simulink model "KT_Robot_Robustness"  (R2025b)
settings: Solver=FixedStepDiscrete  StartTime=0.0  StopTime=tEnd  FixedStep=Ts  RelTol=1e-3
model workspace (MAT data in the model file):
  Ts = 0.05
  impact = [0; 0.1; 0.174532925199; 4; 1; 0.4; 0.04; -0.04; 2; 3.5]
  initialPose = [0; -0.6; 0]
  noise = [-0.649013765191 1.18116604197 -0.758453297284 -1.1096130385 -0.845551240008 -0.572664866458 -0.558680764474 0.17838022585 -0.196861446476 0.586442621667 -0.851886969622 0.800320709802 ... (7323 elements, 3x2441)]
  pathData = [0  0  0  4; 4  0  4  3; 4  3  7  4; 8  3  11  3; 8  6  14  0]
  robot = [0.05; 0.3; 12; 2]
  settings = [0.55; 0.5; 0.05; 1; 1.308996939; 2; 0; 0.12; 0.05; 2400]
  tEnd = 122
(part 1 of 2)
settings Model: Creator=ADMIN  LastModifiedBy=ADMIN
settings DataIOCC: SaveOutput=off  SaveTime=off

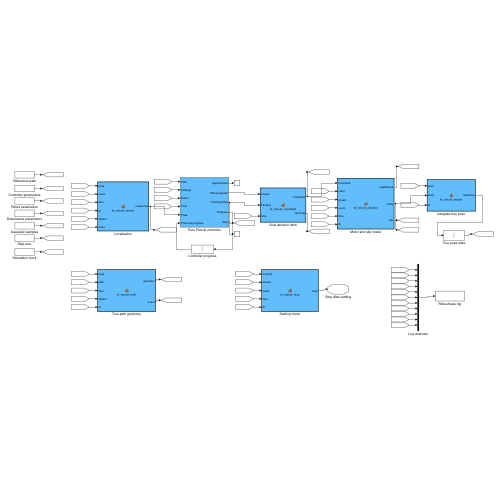
[thumbnail: Simulink's stored preview of the top-level diagram]
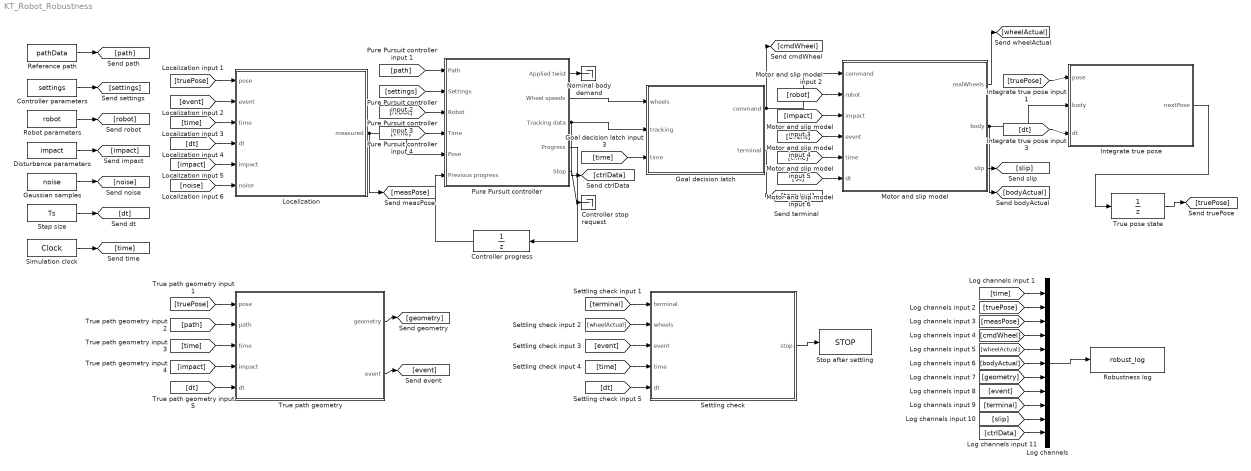
== system KT_Robot_Robustness ==
  Controller parameters : Constant  Value=settings
  Controller progress : UnitDelay  SampleTime=Ts  HasFrameUpgradeWarning=on
  Controller stop request : Terminator
  Disturbance parameters : Constant  Value=impact
  Gaussian samples : Constant  Value=noise
  Goal decision latch : MATLAB Function  TreatAsAtomicUnit=on
  Integrate true pose : MATLAB Function  TreatAsAtomicUnit=on
  Localization : MATLAB Function  TreatAsAtomicUnit=on
  Log channels : Mux  Inputs=[1 3 3 2 2 3 3 3 2 2 6]
  Motor and slip model : MATLAB Function  TreatAsAtomicUnit=on
  Nominal body demand : Terminator
  Pure Pursuit controller : Subsystem
  Reference path : Constant  Value=pathData
  Robot parameters : Constant  Value=robot
  Robustness log : ToWorkspace  VariableName=robust_log  SampleTime=-1
  Settling check : MATLAB Function  TreatAsAtomicUnit=on
  Simulation clock : DigitalClock  SampleTime=Ts
  Step size : Constant  Value=Ts
  Stop after settling : Stop
  True path geometry : MATLAB Function  TreatAsAtomicUnit=on
  True pose state : UnitDelay  InitialCondition=initialPose  SampleTime=Ts  HasFrameUpgradeWarning=on
  wires:
  Reference path/1 -> [path]
  Controller parameters/1 -> [settings]
  Robot parameters/1 -> [robot]
  Disturbance parameters/1 -> [impact]
  Gaussian samples/1 -> [noise]
  Step size/1 -> [dt]
  Simulation clock/1 -> [time]
  Localization/1(measured) -> Pure Pursuit controller/5(Pose), [measPose]
  Pure Pursuit controller/2(Wheel speeds) -> Goal decision latch/1(wheels)
  Pure Pursuit controller/3(Tracking data) -> Goal decision latch/2(tracking), [ctrlData]
  Pure Pursuit controller/1(Applied twist) -> Nominal body demand/1
  Pure Pursuit controller/5(Stop) -> Controller stop request/1
  Pure Pursuit controller/4(Progress) -> Controller progress/1
  Controller progress/1 -> Pure Pursuit controller/6(Previous progress)
  Goal decision latch/1(command) -> Motor and slip model/1(command), [cmdWheel]
  Motor and slip model/2(body) -> Integrate true pose/2(body), [bodyActual]
  Integrate true pose/1(nextPose) -> True pose state/1
  Settling check/1(stop) -> Stop after settling/1
  True pose state/1 -> [truePose]
  True path geometry/1(geometry) -> [geometry]
  True path geometry/2(event) -> [event]
  Goal decision latch/2(terminal) -> [terminal]
  Motor and slip model/1(realWheels) -> [wheelActual]
  Motor and slip model/3(slip) -> [slip]
  [truePose] -> Localization/1(pose)
  [event] -> Localization/2(event)
  [time] -> Localization/3(time)
  [dt] -> Localization/4(dt)
  [impact] -> Localization/5(impact)
  [noise] -> Localization/6(noise)
  [path] -> Pure Pursuit controller/1(Path)
  [settings] -> Pure Pursuit controller/2(Settings)
  [robot] -> Pure Pursuit controller/3(Robot)
  [time] -> Pure Pursuit controller/4(Time)
  [time] -> Goal decision latch/3(time)
  [robot] -> Motor and slip model/2(robot)
  [impact] -> Motor and slip model/3(impact)
  [event] -> Motor and slip model/4(event)
  [time] -> Motor and slip model/5(time)
  [dt] -> Motor and slip model/6(dt)
  [truePose] -> Integrate true pose/1(pose)
  [dt] -> Integrate true pose/3(dt)
  [truePose] -> True path geometry/1(pose)
  [path] -> True path geometry/2(path)
  [time] -> True path geometry/3(time)
  [impact] -> True path geometry/4(impact)
  [dt] -> True path geometry/5(dt)
  [terminal] -> Settling check/1(terminal)
  [wheelActual] -> Settling check/2(wheels)
  [event] -> Settling check/3(event)
  [time] -> Settling check/4(time)
  [dt] -> Settling check/5(dt)
  [time] -> Log channels/1
  [truePose] -> Log channels/2
  [measPose] -> Log channels/3
  [cmdWheel] -> Log channels/4
  [wheelActual] -> Log channels/5
  [bodyActual] -> Log channels/6
  [geometry] -> Log channels/7
  [event] -> Log channels/8
  [terminal] -> Log channels/9
  [slip] -> Log channels/10
  [ctrlData] -> Log channels/11
  Log channels/1 -> Robustness log/1
